simulink model "AirplaneSimModel_SITL"  (R2018b)
settings: Solver=ode2  StartTime=0.0  StopTime=inf  FixedStep=0.0025  RelTol=1e-3
undefined symbols (not defined in the file): aileron_left, aileron_right, airplane, alt_ground, atmosphere, elevator, envir, g, htp_trim, rudder, throttle, wind
libraries: unit_conversions_lib x4, flightgear_visualization_lib x2, ardupilot_sitl_lib x2, conventional_airplane_single_engine_lib x1, atmosphere_lib x1, axes_transformation_lib x1, sensors_lib x1, simulink x1
settings Model: PacingRate=0.500000  Creator=Yannic  LastModifiedBy=yannic
settings OptimizationCC: EfficientMapNaN2IntZero=off
settings HardwareCC: TargetBitPerLong=64  TargetBitPerPointer=64  TargetBitPerSizeT=64  TargetBitPerPtrDiffT=64  TargetLongLongMode=on  TargetIntDivRoundTo=Zero  TargetEndianess=LittleEndian  TargetWordSize=64  TargetHWDeviceType=MATLAB Host  ProdEqTarget=off
settings RTWCC: SystemTargetFile=rsim.tlc  TemplateMakefile=rsim_default_tmf  Description=Rapid Simulation Target  TargetLang=C++  RTWCompilerOptimization=on
settings CodeAppCC: MaxIdLength=128
settings RSimTargetCC: TargetLangStandard=C++03 (ISO)  GeneratePreprocessorConditionals=Use local settings  PreserveStateflowLocalDataDimensions=off

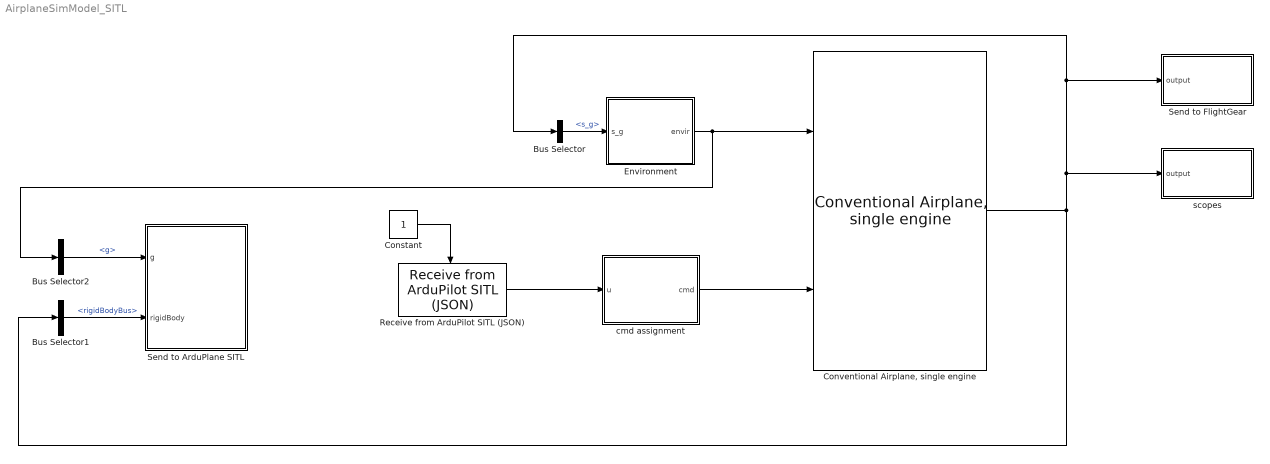
== system AirplaneSimModel_SITL ==
  Bus Selector : BusSelector  OutputSignals=rigidBodyBus.s_g
  Bus Selector1 : BusSelector  OutputSignals=rigidBodyBus
  Bus Selector2 : BusSelector  OutputSignals=g
  Constant : Constant
  "Conventional Airplane, single engine" : conventional_airplane_single_engine_lib/Conventional Airplane, single engine  airplane=airplane
      settings: SourceProductName=LADAC
  Environment : Subsystem
  Receive from ArduPilot SITL (JSON) : ardupilot_sitl_lib/Receive from ArduPilot SITL (JSON)  idx=channel_idx  IP='127.0.0.1'  Port=9002  blocking_time=1
      settings: SourceProductName=LADAC
  Send to ArduPlane SITL : Subsystem
  Send to FlightGear : Subsystem
  cmd assignment : Subsystem
  scopes : Subsystem
  wires:
  Environment/1(envir) -> Bus Selector2/1, "Conventional Airplane, single engine"/1
  "Conventional Airplane, single engine"/1 -> Bus Selector1/1, Bus Selector/1, Send to FlightGear/1(output), scopes/1(output)
  Bus Selector/1 -> Environment/1(s_g)  "<s_g>"
  Bus Selector1/1 -> Send to ArduPlane SITL/2(rigidBody)  "<rigidBodyBus>"
  Bus Selector2/1 -> Send to ArduPlane SITL/1(g)  "<g>"
  cmd assignment/1(cmd) -> "Conventional Airplane, single engine"/2
  Constant/1 -> Receive from ArduPilot SITL (JSON)/Enable
  Receive from ArduPilot SITL (JSON)/1 -> cmd assignment/1(u)

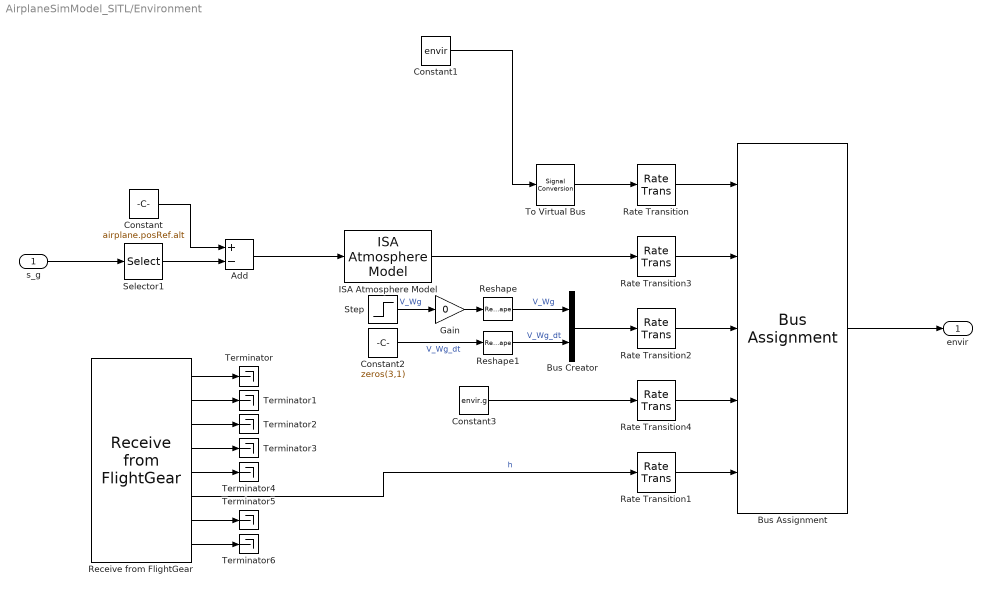
== system AirplaneSimModel_SITL/Environment ==
  s_g : Inport
  Add : Sum  Inputs=+-
  Bus Assignment : BusAssignment  AssignedSignals=atmosphere,wind,g,alt_ground
  Bus Creator : BusCreator  Inputs=2
  Constant : Constant  Value=airplane.posRef.alt
  Constant1 : Constant  Value=envir  OutDataTypeStr=Bus: envirBus
  Constant2 : Constant  Value=zeros(3,1)
  Constant3 : Constant  Value=envir.g
  Gain : Gain  Gain=0
  ISA Atmosphere Model : atmosphere_lib/ISA Atmosphere Model
      settings: SourceProductName=LADAC
  Rate Transition{,1..4} (5 alike) : RateTransition
  Receive from FlightGear : flightgear_visualization_lib/Receive from FlightGear  ip_address='127.0.0.1'  ip_port=5503  sample_time=1/40  blocking_time=0  is_aerocntrl=off  is_engine=off  is_fuel=off  is_land=off  is_avionics=off  is_envir=on
      settings: SourceProductName=LADAC
  Reshape : Reshape  OutputDimensionality=Column vector (2-D)
  Reshape1 : Reshape  OutputDimensionality=Column vector (2-D)
  Selector1 : Selector  InputPortWidth=3  IndexOptions=Index vector (dialog)  Indices=3  OutputSizes=1
  Step : Step  Time=3  After=[0;10;0]  SampleTime=0
  Terminator{,1..6} (7 alike) : Terminator
  To Virtual Bus : SignalConversion  ConversionOutput=Virtual bus  OverrideOpt=off
  envir : Outport
  wires:
  Receive from FlightGear/6 -> Rate Transition1/1  "h"
  Rate Transition2/1 -> Bus Assignment/3
  Rate Transition3/1 -> Bus Assignment/2
  Bus Assignment/1 -> envir/1
  Rate Transition/1 -> Bus Assignment/1
  ISA Atmosphere Model/1 -> Rate Transition3/1
  Step/1 -> Gain/1  "V_Wg"
  Rate Transition1/1 -> Bus Assignment/5
  s_g/1 -> Selector1/1
  Bus Creator/1 -> Rate Transition2/1
  Constant2/1 -> Reshape1/1  "V_Wg_dt"
  Rate Transition4/1 -> Bus Assignment/4
  Constant3/1 -> Rate Transition4/1
  Gain/1 -> Reshape/1
  Constant/1 -> Add/1
  Add/1 -> ISA Atmosphere Model/1
  Selector1/1 -> Add/2
  To Virtual Bus/1 -> Rate Transition/1
  Reshape/1 -> Bus Creator/1  "V_Wg"
  Reshape1/1 -> Bus Creator/2  "V_Wg_dt"
  Constant1/1 -> To Virtual Bus/1
  Receive from FlightGear/1 -> Terminator/1
  Receive from FlightGear/2 -> Terminator1/1
  Receive from FlightGear/3 -> Terminator2/1
  Receive from FlightGear/4 -> Terminator3/1
  Receive from FlightGear/5 -> Terminator4/1
  Receive from FlightGear/7 -> Terminator5/1
  Receive from FlightGear/8 -> Terminator6/1

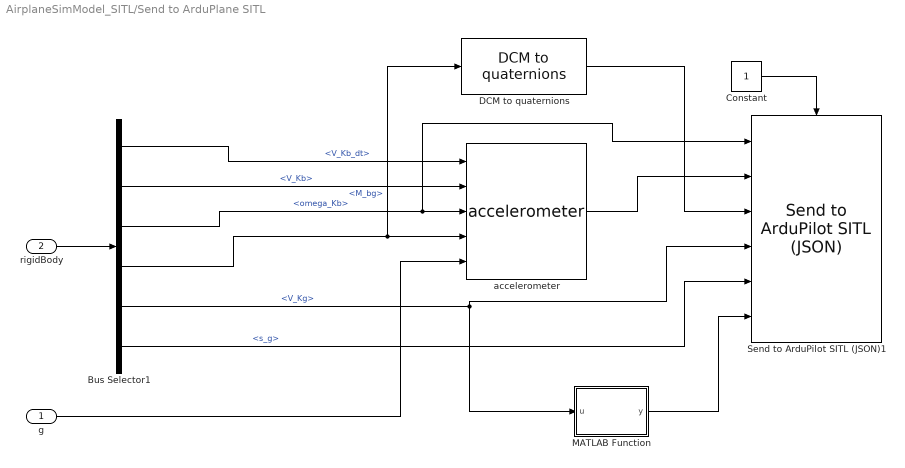
== system AirplaneSimModel_SITL/Send to ArduPlane SITL ==
  g : Inport
  rigidBody : Inport  Port=2
  Bus Selector1 : BusSelector  OutputSignals=V_Kb_dt,V_Kb,omega_Kb,M_bg,V_Kg,s_g
  Constant : Constant
  DCM to quaternions : axes_transformation_lib/DCM to quaternions  SystemSampleTime=-1
      settings: SourceProductName=LADAC
  MATLAB Function : MATLAB Function  TreatAsAtomicUnit=on
  Send to ArduPilot SITL (JSON)1 : ardupilot_sitl_lib/Send to ArduPilot SITL (JSON)  IP='127.0.0.1'  Port=9003  sample_time=1/400  opt_signals_str="'\"airplane\":%f'"  ap_rot=[0;0;pi]
      settings: SourceProductName=LADAC
  accelerometer : sensors_lib/accelerometer  SystemSampleTime=-1
      settings: SourceProductName=LADAC
  wires:
  g/1 -> accelerometer/5
  rigidBody/1 -> Bus Selector1/1
  Constant/1 -> Send to ArduPilot SITL (JSON)1/Enable
  accelerometer/1 -> Send to ArduPilot SITL (JSON)1/2
  Bus Selector1/6 -> Send to ArduPilot SITL (JSON)1/5  "<s_g>"
  Bus Selector1/5 -> Send to ArduPilot SITL (JSON)1/4, MATLAB Function/1(u)  "<V_Kg>"
  MATLAB Function/1(y) -> Send to ArduPilot SITL (JSON)1/6
  Bus Selector1/1 -> accelerometer/1  "<V_Kb_dt>"
  Bus Selector1/2 -> accelerometer/2  "<V_Kb>"
  Bus Selector1/3 -> Send to ArduPilot SITL (JSON)1/1, accelerometer/3  "<omega_Kb>"
  Bus Selector1/4 -> DCM to quaternions/1, accelerometer/4  "<M_bg>"
  DCM to quaternions/1 -> Send to ArduPilot SITL (JSON)1/3

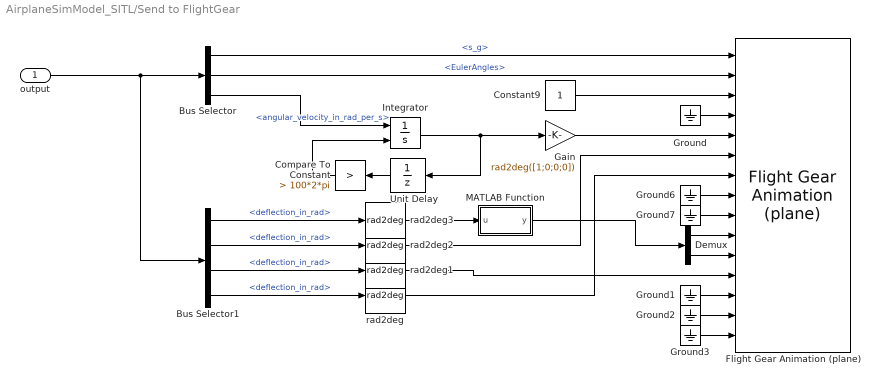
== system AirplaneSimModel_SITL/Send to FlightGear ==
  output : Inport
  Bus Selector : BusSelector  OutputSignals=rigidBodyBus.s_g,rigidBodyBus.EulerAngles,actuatorBus.motorBus.angular_velocity_in_rad_per_s
  Bus Selector1 : BusSelector  OutputSignals=actuatorBus.aileronsBus.deflection_in_rad,actuatorBus.elevatorBus.deflection_in_rad,actuatorBus.rudderBus.deflection_in_rad,actuatorBus.htpTrimBus.deflection_in_rad
  Compare To Constant : simulink/Logic and Bit Operations/Compare To Constant  relop=>  const=100*2*pi  OutDataTypeStr=boolean
  Constant9 : Constant
  Demux : Demux  Outputs=2
  Flight Gear Animation (plane) : flightgear_visualization_lib/Flight Gear Animation (plane)  inital_lat=airplane.posRef.lat  inital_long=airplane.posRef.lon  inital_height=airplane.posRef.alt  remoteURL='127.0.0.1'  remotePort=5502
      settings: SourceProductName=LADAC
  Gain : Gain  Gain=rad2deg([1;0;0;0])
  Ground{,1..3,6..7} (6 alike) : Ground
  Integrator : Integrator  ExternalReset=rising
  MATLAB Function : MATLAB Function  TreatAsAtomicUnit=on
  Unit Delay : UnitDelay  SampleTime=-1
  rad2deg{,1..3} (4 alike) : unit_conversions_lib/rad2deg
      settings: SourceProductName=LADAC
  wires:
  Compare To Constant/1 -> Integrator/2
  Integrator/1 -> Unit Delay/1, Gain/1
  Bus Selector/1 -> Flight Gear Animation (plane)/1  "<s_g>"
  Bus Selector/2 -> Flight Gear Animation (plane)/2  "<EulerAngles>"
  Gain/1 -> Flight Gear Animation (plane)/5
  Constant9/1 -> Flight Gear Animation (plane)/3
  Unit Delay/1 -> Compare To Constant/1
  Ground/1 -> Flight Gear Animation (plane)/4
  Ground1/1 -> Flight Gear Animation (plane)/13
  Ground2/1 -> Flight Gear Animation (plane)/14
  Ground3/1 -> Flight Gear Animation (plane)/15
  output/1 -> Bus Selector1/1, Bus Selector/1
  Bus Selector/3 -> Integrator/1  "<angular_velocity_in_rad_per_s>"
  Bus Selector1/2 -> rad2deg2/1  "<deflection_in_rad>"
  Bus Selector1/4 -> rad2deg/1  "<deflection_in_rad>"
  Ground6/1 -> Flight Gear Animation (plane)/8
  Ground7/1 -> Flight Gear Animation (plane)/9
  Bus Selector1/3 -> rad2deg1/1  "<deflection_in_rad>"
  Bus Selector1/1 -> rad2deg3/1  "<deflection_in_rad>"
  Demux/1 -> Flight Gear Animation (plane)/10
  Demux/2 -> Flight Gear Animation (plane)/11
  rad2deg/1 -> Flight Gear Animation (plane)/7
  rad2deg1/1 -> Flight Gear Animation (plane)/12
  rad2deg2/1 -> Flight Gear Animation (plane)/6
  rad2deg3/1 -> MATLAB Function/1(u)
  MATLAB Function/1(y) -> Demux/1

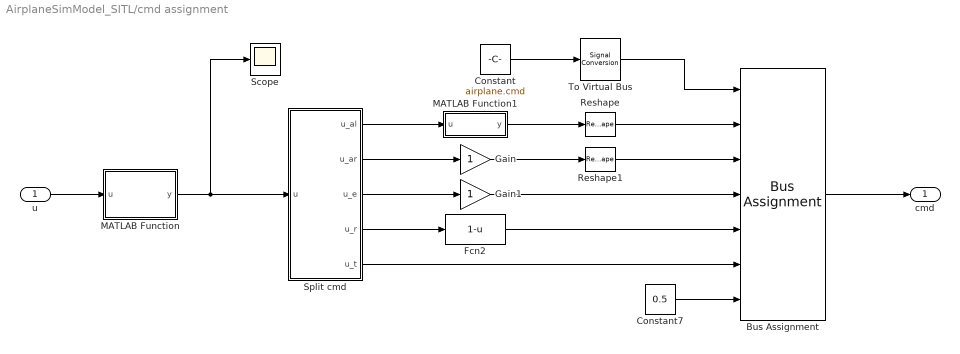
== system AirplaneSimModel_SITL/cmd assignment ==
  u : Inport
  Bus Assignment : BusAssignment  AssignedSignals=aileron_left,aileron_right,elevator,rudder,throttle,htp_trim
  Constant : Constant  Value=airplane.cmd  OutDataTypeStr=Bus: cmdBus
  Constant7 : Constant  Value=0.5
  Fcn2 : Fcn  Expr=1-u
  Gain : Gain
  Gain1 : Gain
  MATLAB Function : MATLAB Function  TreatAsAtomicUnit=on
  MATLAB Function1 : MATLAB Function  TreatAsAtomicUnit=on
  Reshape : Reshape  OutputDimensionality=Row vector (2-D)
  Reshape1 : Reshape  OutputDimensionality=Row vector (2-D)
  Scope : Scope
  Split cmd : MATLAB Function  TreatAsAtomicUnit=on
  To Virtual Bus : SignalConversion  ConversionOutput=Virtual bus  OverrideOpt=off
  cmd : Outport
  wires:
  Constant/1 -> To Virtual Bus/1
  Bus Assignment/1 -> cmd/1
  Constant7/1 -> Bus Assignment/7
  u/1 -> MATLAB Function/1(u)
  Split cmd/5(u_t) -> Bus Assignment/6
  Split cmd/3(u_e) -> Gain1/1
  Split cmd/4(u_r) -> Fcn2/1
  To Virtual Bus/1 -> Bus Assignment/1
  Gain/1 -> Reshape1/1
  MATLAB Function1/1(y) -> Reshape/1
  Gain1/1 -> Bus Assignment/4
  Fcn2/1 -> Bus Assignment/5
  MATLAB Function/1(y) -> Scope/1, Split cmd/1(u)
  Split cmd/2(u_ar) -> Gain/1
  Split cmd/1(u_al) -> MATLAB Function1/1(u)
  Reshape/1 -> Bus Assignment/2
  Reshape1/1 -> Bus Assignment/3

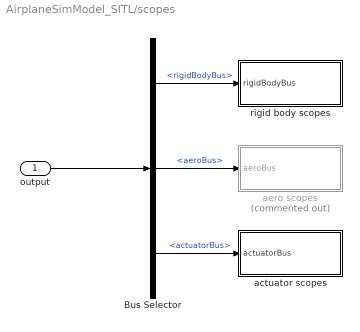
== system AirplaneSimModel_SITL/scopes ==
  output : Inport
  Bus Selector : BusSelector  OutputSignals=rigidBodyBus,aeroBus,actuatorBus
  actuator scopes : Subsystem
  aero scopes : Subsystem  Commented=on
  rigid body scopes : Subsystem
  wires:
  Bus Selector/1 -> rigid body scopes/1(rigidBodyBus)  "<rigidBodyBus>"
  Bus Selector/2 -> aero scopes/1(aeroBus)  "<aeroBus>"
  output/1 -> Bus Selector/1
  Bus Selector/3 -> actuator scopes/1(actuatorBus)  "<actuatorBus>"

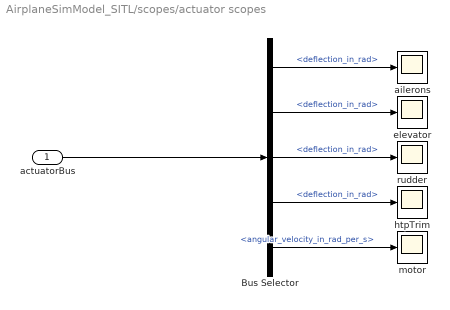
== system AirplaneSimModel_SITL/scopes/actuator scopes ==
  actuatorBus : Inport
  Bus Selector : BusSelector  OutputSignals=aileronsBus.deflection_in_rad,elevatorBus.deflection_in_rad,rudderBus.deflection_in_rad,htpTrimBus.deflection_in_rad,motorBus.angular_velocity_in_rad_per_s
  ailerons : Scope
  elevator : Scope
  htpTrim : Scope
  motor : Scope
  rudder : Scope
  wires:
  actuatorBus/1 -> Bus Selector/1
  Bus Selector/1 -> ailerons/1  "<deflection_in_rad>"
  Bus Selector/2 -> elevator/1  "<deflection_in_rad>"
  Bus Selector/3 -> rudder/1  "<deflection_in_rad>"
  Bus Selector/4 -> htpTrim/1  "<deflection_in_rad>"
  Bus Selector/5 -> motor/1  "<angular_velocity_in_rad_per_s>"

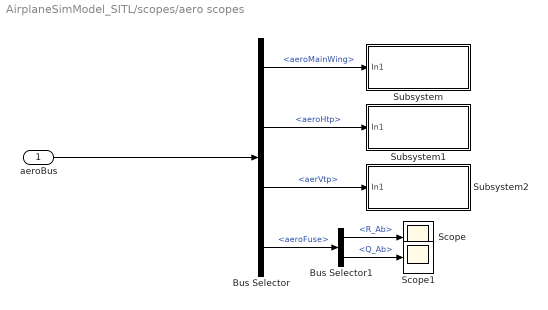
== system AirplaneSimModel_SITL/scopes/aero scopes ==
  aeroBus : Inport
  Bus Selector : BusSelector  OutputSignals=aeroMainWing,aeroHtp,aerVtp,aeroFuse
  Bus Selector1 : BusSelector  OutputSignals=R_Ab,Q_Ab
  Scope : Scope
  Scope1 : Scope
  Subsystem : Subsystem
  Subsystem1 : Subsystem
  Subsystem2 : Subsystem
  wires:
  aeroBus/1 -> Bus Selector/1
  Bus Selector/1 -> Subsystem/1(In1)  "<aeroMainWing>"
  Bus Selector/2 -> Subsystem1/1(In1)  "<aeroHtp>"
  Bus Selector/3 -> Subsystem2/1(In1)  "<aerVtp>"
  Bus Selector/4 -> Bus Selector1/1  "<aeroFuse>"
  Bus Selector1/1 -> Scope/1  "<R_Ab>"
  Bus Selector1/2 -> Scope1/1  "<Q_Ab>"

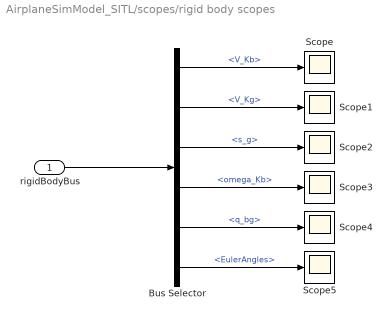
== system AirplaneSimModel_SITL/scopes/rigid body scopes ==
  rigidBodyBus : Inport
  Bus Selector : BusSelector  OutputSignals=V_Kb,V_Kg,s_g,omega_Kb,q_bg,EulerAngles
  Scope{,1..5} (6 alike) : Scope
  wires:
  rigidBodyBus/1 -> Bus Selector/1
  Bus Selector/1 -> Scope/1  "<V_Kb>"
  Bus Selector/2 -> Scope1/1  "<V_Kg>"
  Bus Selector/3 -> Scope2/1  "<s_g>"
  Bus Selector/4 -> Scope3/1  "<omega_Kb>"
  Bus Selector/5 -> Scope4/1  "<q_bg>"
  Bus Selector/6 -> Scope5/1  "<EulerAngles>"

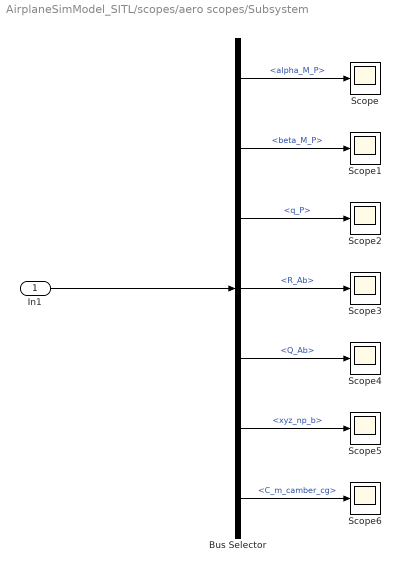
== system AirplaneSimModel_SITL/scopes/aero scopes/Subsystem ==
  In1 : Inport
  Bus Selector : BusSelector  OutputSignals=aeroAxes.alpha_M_P,aeroAxes.beta_M_P,aeroAxes.q_P,dynamics.R_Ab,dynamics.Q_Ab,dynamics.xyz_np_b,dynamics.C_m_camber_cg
  Scope{,1..6} (7 alike) : Scope
  wires:
  In1/1 -> Bus Selector/1
  Bus Selector/1 -> Scope/1  "<alpha_M_P>"
  Bus Selector/3 -> Scope2/1  "<q_P>"
  Bus Selector/2 -> Scope1/1  "<beta_M_P>"
  Bus Selector/4 -> Scope3/1  "<R_Ab>"
  Bus Selector/5 -> Scope4/1  "<Q_Ab>"
  Bus Selector/6 -> Scope5/1  "<xyz_np_b>"
  Bus Selector/7 -> Scope6/1  "<C_m_camber_cg>"

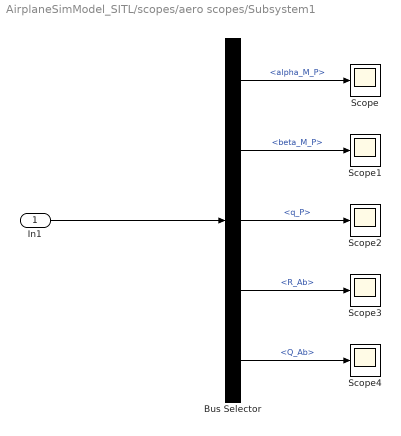
== system AirplaneSimModel_SITL/scopes/aero scopes/Subsystem1 ==
  In1 : Inport
  Bus Selector : BusSelector  OutputSignals=aeroAxes.alpha_M_P,aeroAxes.beta_M_P,aeroAxes.q_P,dynamics.R_Ab,dynamics.Q_Ab
  Scope{,1..4} (5 alike) : Scope
  wires:
  Bus Selector/5 -> Scope4/1  "<Q_Ab>"
  Bus Selector/4 -> Scope3/1  "<R_Ab>"
  Bus Selector/2 -> Scope1/1  "<beta_M_P>"
  Bus Selector/3 -> Scope2/1  "<q_P>"
  Bus Selector/1 -> Scope/1  "<alpha_M_P>"
  In1/1 -> Bus Selector/1

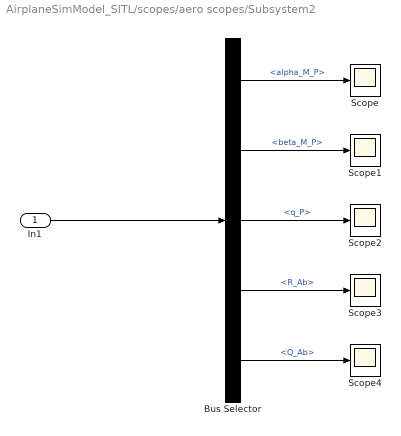
== system AirplaneSimModel_SITL/scopes/aero scopes/Subsystem2 ==
  In1 : Inport
  Bus Selector : BusSelector  OutputSignals=aeroAxes.alpha_M_P,aeroAxes.beta_M_P,aeroAxes.q_P,dynamicsBody.R_Ab,dynamicsBody.Q_Ab
  Scope{,1..4} (5 alike) : Scope
  wires:
  In1/1 -> Bus Selector/1
  Bus Selector/1 -> Scope/1  "<alpha_M_P>"
  Bus Selector/3 -> Scope2/1  "<q_P>"
  Bus Selector/2 -> Scope1/1  "<beta_M_P>"
  Bus Selector/4 -> Scope3/1  "<R_Ab>"
  Bus Selector/5 -> Scope4/1  "<Q_Ab>"

== matlab function AirplaneSimModel_SITL/cmd assignment/MATLAB Function1 ==
  data: u input; y output
function y = fcn(u)
y = 1 - u;
end

== matlab function AirplaneSimModel_SITL/Send to ArduPlane SITL/MATLAB Function ==
  data: u input; y output
function y = fcn(u)

y = norm(u,2);

== matlab function AirplaneSimModel_SITL/Send to FlightGear/MATLAB Function ==
  data: u input; y output
function y = fcn(u)
y = u([1,end]);
end

== matlab function AirplaneSimModel_SITL/cmd assignment/MATLAB Function ==
  data: u input; y output
function y = fcn(u)

y = (u-0.1)/0.8;

== matlab function AirplaneSimModel_SITL/cmd assignment/Split cmd ==
  data: u input; u_al output; u_ar output; u_e output; u_r output; u_t output
function [u_al,u_ar,u_e,u_r,u_t] = fcn(u)
n_a = (length(u)-3)/2;
u_al = u(1:n_a);
u_ar = u(n_a+1:2*n_a);
u_e = u(end-2);
u_r = u(end-1);
u_t = u(end);
end
